simulink library "fmCopterLoiterIndi_lib"  (R2018b)
settings: Solver=VariableStepAuto  StartTime=0.0  StopTime=10.0  RelTol=1e-3
undefined symbols (not defined in the file or in its folder): fm_loiter
libraries: filters_lib x5, indi_lib x3, cntrlAttiRedIndi_lib x1, cntrlPosNdi_lib x1
settings Model: Creator=Ybeyer  LastModifiedBy=yannic
settings SFSimCC: SimUseLocalCustomCode=off
settings RTWCC: RTWUseLocalCustomCode=off
settings CodeAppCC: StateflowObjectComments=on

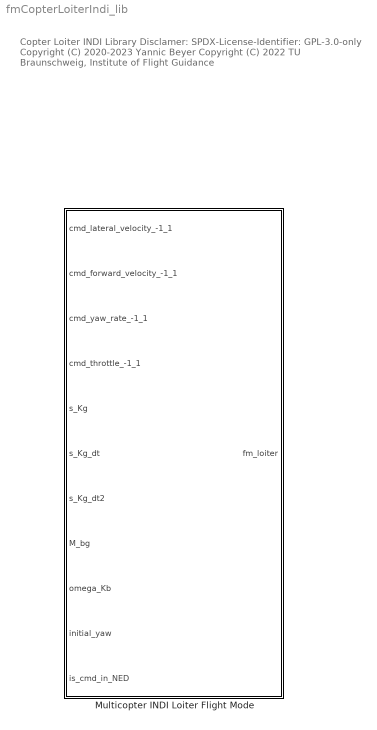
== system fmCopterLoiterIndi_lib ==
  note: Copter Loiter INDI Library
      |
      | Disclamer:
      | SPDX-License-Identifier: GPL-3.0-only
      |
      | Copyright (C) 2020-2023 Yannic Beyer
      | Copyright (C) 2022 TU Braunschweig, Institute of Flight Guidance
  Multicopter INDI Loiter Flight Mode : Subsystem  mask{fm=fm_loiter}
      mask prompts: fm "Copter INDI loiter flight mode parameters struct, see fmCopterLoiterIndi_params_default"
      mask DialogControl DescGroupVar Prompt: Multicopter INDI Loiter Flight Mode
      mask DialogControl DescTextVar Prompt: Loiter flight mode using the reduced attitude controller with INDI.

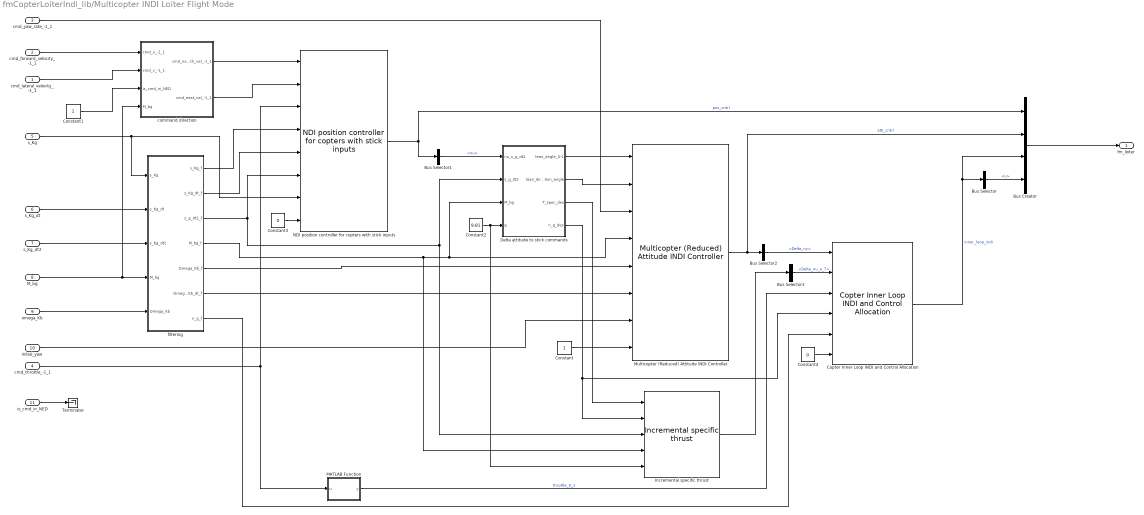
== system fmCopterLoiterIndi_lib/Multicopter INDI Loiter Flight Mode ==
  cmd_lateral_velocity_-1_1 : Inport  SampleTime=fm.ts
  cmd_forward_velocity_-1_1 : Inport  Port=2  SampleTime=fm.ts
  cmd_yaw_rate_-1_1 : Inport  Port=3  SampleTime=fm.ts
  cmd_throttle_-1_1 : Inport  Port=4  SampleTime=fm.ts
  s_Kg : Inport  Port=5  SampleTime=fm.ts
  s_Kg_dt : Inport  Port=6  SampleTime=fm.ts
  s_Kg_dt2 : Inport  Port=7  SampleTime=fm.ts
  M_bg : Inport  Port=8  SampleTime=fm.ts
  omega_Kb : Inport  Port=9  SampleTime=fm.ts
  initial_yaw : Inport  Port=10  SampleTime=fm.ts
  is_cmd_in_NED : Inport  Port=11  SampleTime=fm.ts
  Bus Creator : BusCreator  Inputs=4
  Bus Selector : BusSelector  OutputSignals=u
  Bus Selector1 : BusSelector  OutputSignals=pseudo_control.nu
  Bus Selector2 : BusSelector  OutputSignals=pseudo_control.Delta_ny
  Bus Selector3 : BusSelector  OutputSignals=Delta_nu_a_T
  Constant : Constant
  Constant1 : Constant
  Constant2 : Constant  Value=9.81
  Constant3 : Constant  Value=0
  Constant4 : Constant  Value=0
  Copter Inner Loop INDI and Control Allocation : indi_lib/Copter Inner Loop INDI and Control Allocation  cep=fm.cep  ceb=fm.ceb  ca=fm.ca  mtc=fm.mtc  sflt=fm.sflt  ts=fm.ts
      settings: SourceProductName=LADAC
  Delta attitude to stick commands : Subsystem
  Incremental specific thrust : indi_lib/Incremental specific thrust  leanfreq=fm.atc.rm.leanfreq  leandamp=fm.atc.rm.leandamp  is_enable_checked=off  states_when_enabling=held
      settings: SourceProductName=LADAC
  MATLAB Function : MATLAB Function  TreatAsAtomicUnit=on
  Multicopter (Reduced) Attitude INDI Controller : cntrlAttiRedIndi_lib/Multicopter (Reduced) Attitude INDI Controller  atc=fm.atc  T=fm.mtc + 2./fm.sflt.omega
      settings: SourceProductName=LADAC
  NDI position controller for copters with stick inputs : cntrlPosNdi_lib/NDI position controller for copters with stick inputs  psc=fm.psc  T_inner_loop=2./fm.atc.rm.leanfreq + fm.mtc + 2./fm.sflt.omega  is_enable_checked=off  states_when_enabling=held
      settings: SourceProductName=LADAC
  Terminator : Terminator
  command direction : Subsystem
  filtering : Subsystem
  fm_loiter : Outport  SampleTime=fm.ts
  wires:
  cmd_forward_velocity_-1_1/1 -> command direction/1(cmd_u_-1_1)
  filtering/2(s_Kg_dt_f) -> NDI position controller for copters with stick inputs/5
  filtering/3(s_g_dt2_f) -> NDI position controller for copters with stick inputs/6, Incremental specific thrust/3, Delta attitude to stick commands/2(s_g_dt2)
  cmd_yaw_rate_-1_1/1 -> Multicopter (Reduced) Attitude INDI Controller/3
  Constant/1 -> Multicopter (Reduced) Attitude INDI Controller/8
  filtering/1(s_Kg_f) -> NDI position controller for copters with stick inputs/4
  filtering/5(Omega_Kb_f) -> Multicopter (Reduced) Attitude INDI Controller/5
  NDI position controller for copters with stick inputs/1 -> Bus Creator/1, Bus Selector1/1  "pos_cntrl"
  filtering/4(M_bg_f) -> Incremental specific thrust/4, Multicopter (Reduced) Attitude INDI Controller/4, Delta attitude to stick commands/3(M_bg)
  initial_yaw/1 -> Multicopter (Reduced) Attitude INDI Controller/7
  cmd_lateral_velocity_-1_1/1 -> command direction/2(cmd_v_-1_1)
  Constant1/1 -> command direction/3(is_cmd_in_NED)
  Bus Selector1/1 -> Delta attitude to stick commands/1(nu_s_g_dt2)  "<nu>"
  Bus Creator/1 -> fm_loiter/1
  command direction/1(cmd_north_vel_-1_1) -> NDI position controller for copters with stick inputs/1
  command direction/2(cmd_east_vel_-1_1) -> NDI position controller for copters with stick inputs/2
  is_cmd_in_NED/1 -> Terminator/1
  Multicopter (Reduced) Attitude INDI Controller/1 -> Bus Selector2/1, Bus Creator/2  "atti_cntrl"
  filtering/6(Omega_Kb_dt_f) -> Multicopter (Reduced) Attitude INDI Controller/6
  Delta attitude to stick commands/2(lean_direction_angle) -> Multicopter (Reduced) Attitude INDI Controller/2
  Delta attitude to stick commands/1(lean_angle_0-1) -> Multicopter (Reduced) Attitude INDI Controller/1
  MATLAB Function/1(y) -> Copter Inner Loop INDI and Control Allocation/3  "throttle_0_1"
  Copter Inner Loop INDI and Control Allocation/1 -> Bus Selector/1, Bus Creator/3  "inner_loop_indi"
  cmd_throttle_-1_1/1 -> NDI position controller for copters with stick inputs/3, MATLAB Function/1(u)
  Bus Selector2/1 -> Copter Inner Loop INDI and Control Allocation/1  "<Delta_ny>"
  Constant2/1 -> Incremental specific thrust/5, Delta attitude to stick commands/4(g)
  Bus Selector/1 -> Bus Creator/4  "<u>"
  Incremental specific thrust/1 -> Bus Selector3/1
  Delta attitude to stick commands/3(T_spec_des) -> Incremental specific thrust/1
  Constant3/1 -> NDI position controller for copters with stick inputs/8
  s_Kg/1 -> NDI position controller for copters with stick inputs/7, filtering/1(s_Kg)
  M_bg/1 -> command direction/4(M_bg), filtering/4(M_bg)
  omega_Kb/1 -> filtering/5(Omega_Kb)
  s_Kg_dt2/1 -> filtering/3(s_Kg_dt2)
  s_Kg_dt/1 -> filtering/2(s_Kg_dt)
  filtering/7(n_g_f) -> Copter Inner Loop INDI and Control Allocation/5
  Delta attitude to stick commands/4(n_g_des) -> Copter Inner Loop INDI and Control Allocation/4, Incremental specific thrust/2
  Bus Selector3/1 -> Copter Inner Loop INDI and Control Allocation/2  "<Delta_nu_a_T>"
  Constant4/1 -> Copter Inner Loop INDI and Control Allocation/6

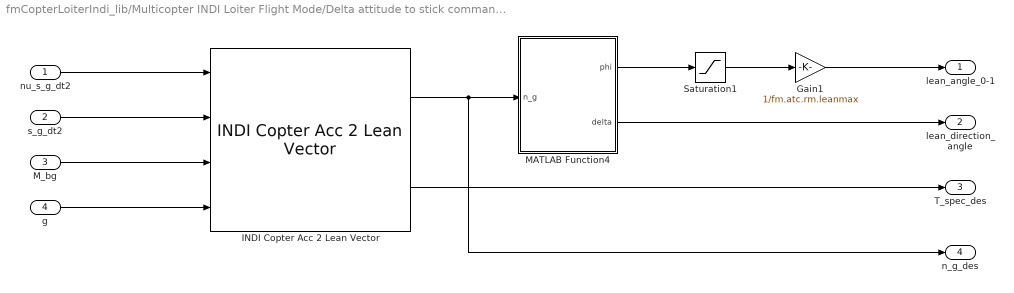
== system fmCopterLoiterIndi_lib/Multicopter INDI Loiter Flight Mode/Delta attitude to stick commands ==
  nu_s_g_dt2 : Inport
  s_g_dt2 : Inport  Port=2
  M_bg : Inport  Port=3
  g : Inport  Port=4
  Gain1 : Gain  Gain=1/fm.atc.rm.leanmax
  INDI Copter Acc 2 Lean Vector : indi_lib/INDI Copter Acc 2 Lean Vector  SystemSampleTime=-1
      settings: SourceProductName=LADAC
  MATLAB Function4 : MATLAB Function  TreatAsAtomicUnit=on
  Saturation1 : Saturate  UpperLimit=fm.atc.rm.leanmax  LowerLimit=0
  lean_angle_0-1 : Outport
  lean_direction_angle : Outport  Port=2
  T_spec_des : Outport  Port=3
  n_g_des : Outport  Port=4
  wires:
  M_bg/1 -> INDI Copter Acc 2 Lean Vector/3
  s_g_dt2/1 -> INDI Copter Acc 2 Lean Vector/2
  g/1 -> INDI Copter Acc 2 Lean Vector/4
  MATLAB Function4/1(phi) -> Saturation1/1
  Saturation1/1 -> Gain1/1
  nu_s_g_dt2/1 -> INDI Copter Acc 2 Lean Vector/1
  Gain1/1 -> lean_angle_0-1/1
  MATLAB Function4/2(delta) -> lean_direction_angle/1
  INDI Copter Acc 2 Lean Vector/1 -> n_g_des/1, MATLAB Function4/1(n_g)
  INDI Copter Acc 2 Lean Vector/2 -> T_spec_des/1

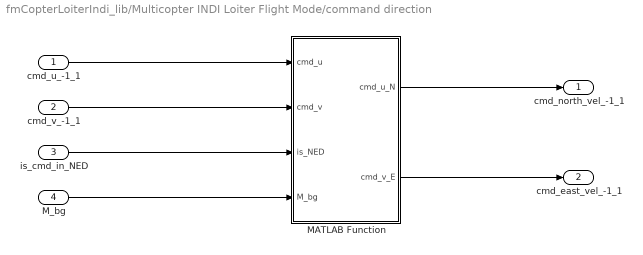
== system fmCopterLoiterIndi_lib/Multicopter INDI Loiter Flight Mode/command direction ==
  cmd_u_-1_1 : Inport
  cmd_v_-1_1 : Inport  Port=2
  is_cmd_in_NED : Inport  Port=3
  M_bg : Inport  Port=4
  MATLAB Function : MATLAB Function  TreatAsAtomicUnit=on
  cmd_north_vel_-1_1 : Outport
  cmd_east_vel_-1_1 : Outport  Port=2
  wires:
  cmd_u_-1_1/1 -> MATLAB Function/1(cmd_u)
  cmd_v_-1_1/1 -> MATLAB Function/2(cmd_v)
  is_cmd_in_NED/1 -> MATLAB Function/3(is_NED)
  MATLAB Function/1(cmd_u_N) -> cmd_north_vel_-1_1/1
  MATLAB Function/2(cmd_v_E) -> cmd_east_vel_-1_1/1
  M_bg/1 -> MATLAB Function/4(M_bg)

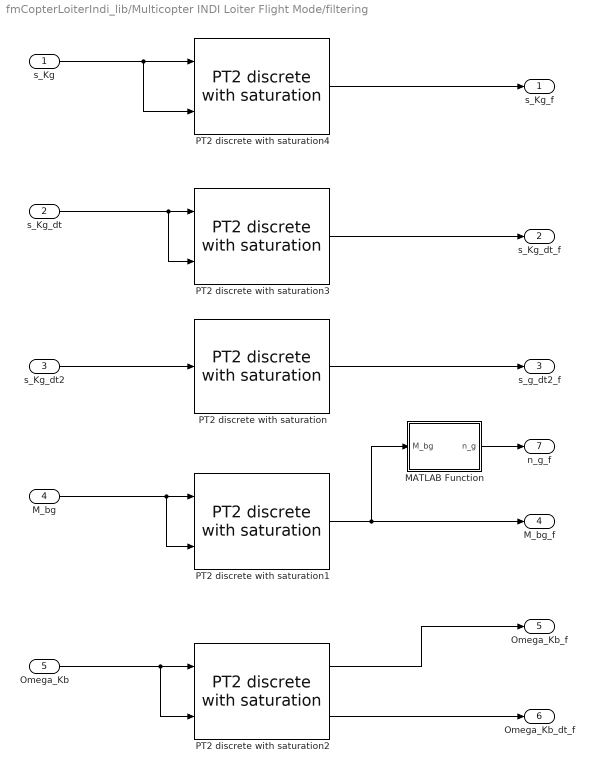
== system fmCopterLoiterIndi_lib/Multicopter INDI Loiter Flight Mode/filtering ==
  s_Kg : Inport
  s_Kg_dt : Inport  Port=2
  s_Kg_dt2 : Inport  Port=3
  M_bg : Inport  Port=4
  Omega_Kb : Inport  Port=5
  MATLAB Function : MATLAB Function  TreatAsAtomicUnit=on
  PT2 discrete with saturation : filters_lib/PT2 discrete with saturation  param_src=internal  omega=fm.sflt.omega  d=fm.sflt.D  x_dt2_max=inf  x_dt2_min=-inf  x_dt_max=inf  x_dt_min=-inf  x_max=inf  x_min=-inf  y_0_src=internal  x_init=0  y_dt_0_src=internal  x_dt_init=0  is_y_dt_checked=off  is_y_dt2_checked=off
      settings: SourceProductName=LADAC
  PT2 discrete with saturation1 : filters_lib/PT2 discrete with saturation  param_src=internal  omega=fm.sflt.omega  d=fm.sflt.D  x_dt2_max=inf  x_dt2_min=-inf  x_dt_max=inf  x_dt_min=-inf  x_max=inf  x_min=-inf  y_0_src=external  x_init=0  y_dt_0_src=internal  x_dt_init=0  is_y_dt_checked=off  is_y_dt2_checked=off
      settings: SourceProductName=LADAC
  PT2 discrete with saturation2 : filters_lib/PT2 discrete with saturation  param_src=internal  omega=fm.sflt.omega  d=fm.sflt.D  x_dt2_max=inf  x_dt2_min=-inf  x_dt_max=inf  x_dt_min=-inf  x_max=inf  x_min=-inf  y_0_src=external  x_init=0  y_dt_0_src=internal  x_dt_init=0  is_y_dt_checked=on  is_y_dt2_checked=off
      settings: SourceProductName=LADAC
  PT2 discrete with saturation3 : filters_lib/PT2 discrete with saturation  param_src=internal  omega=fm.sflt.omega  d=fm.sflt.D  x_dt2_max=inf  x_dt2_min=-inf  x_dt_max=inf  x_dt_min=-inf  x_max=inf  x_min=-inf  y_0_src=external  x_init=0  y_dt_0_src=internal  x_dt_init=0  is_y_dt_checked=off  is_y_dt2_checked=off
      settings: SourceProductName=LADAC
  PT2 discrete with saturation4 : filters_lib/PT2 discrete with saturation  param_src=internal  omega=fm.sflt.omega  d=fm.sflt.D  x_dt2_max=inf  x_dt2_min=-inf  x_dt_max=inf  x_dt_min=-inf  x_max=inf  x_min=-inf  y_0_src=external  x_init=0  y_dt_0_src=internal  x_dt_init=0  is_y_dt_checked=off  is_y_dt2_checked=off
      settings: SourceProductName=LADAC
  s_Kg_f : Outport
  s_Kg_dt_f : Outport  Port=2
  s_g_dt2_f : Outport  Port=3
  M_bg_f : Outport  Port=4
  Omega_Kb_f : Outport  Port=5
  Omega_Kb_dt_f : Outport  Port=6
  n_g_f : Outport  Port=7
  wires:
  PT2 discrete with saturation2/2 -> Omega_Kb_dt_f/1
  Omega_Kb/1 -> PT2 discrete with saturation2/2, PT2 discrete with saturation2/1
  PT2 discrete with saturation2/1 -> Omega_Kb_f/1
  M_bg/1 -> PT2 discrete with saturation1/2, PT2 discrete with saturation1/1
  PT2 discrete with saturation/1 -> s_g_dt2_f/1
  s_Kg_dt2/1 -> PT2 discrete with saturation/1
  PT2 discrete with saturation3/1 -> s_Kg_dt_f/1
  s_Kg_dt/1 -> PT2 discrete with saturation3/2, PT2 discrete with saturation3/1
  PT2 discrete with saturation4/1 -> s_Kg_f/1
  s_Kg/1 -> PT2 discrete with saturation4/1, PT2 discrete with saturation4/2
  PT2 discrete with saturation1/1 -> MATLAB Function/1(M_bg), M_bg_f/1
  MATLAB Function/1(n_g) -> n_g_f/1

== matlab function fmCopterLoiterIndi_lib/Multicopter INDI Loiter Flight Mode/command direction/MATLAB Function ==
  data: cmd_u input; cmd_u_N output; cmd_v input; is_NED input; cmd_v_E output; M_bg input
function [cmd_u_N,cmd_v_E] = fcn( cmd_u, cmd_v, is_NED, M_bg )

if is_NED
    cmd_u_N = cmd_u;
    cmd_v_E = cmd_v;
else
    EulerAngle = dcm2Euler(M_bg);
    yaw = EulerAngle(3);
    M_NED_FRD = euler2Dcm([0;0;yaw])';
    cmd_V_NED = M_NED_FRD * [ cmd_u; cmd_v; 0 ];
    cmd_u_N = cmd_V_NED(1);
    cmd_v_E = cmd_V_NED(2);
end

end

== matlab function fmCopterLoiterIndi_lib/Multicopter INDI Loiter Flight Mode/filtering/MATLAB Function ==
  data: M_bg input; n_g output
function n_g = dcm2LeanVector( M_bg )
n_g = dcm2LeanVector( M_bg );
end

== matlab function fmCopterLoiterIndi_lib/Multicopter INDI Loiter Flight Mode/Delta attitude to stick commands/MATLAB Function4 ==
  data: n_g input; phi output; delta output
function [phi,delta] = leanVector2LeanAngles(n_g)
[phi,delta] = leanVector2LeanAngles(n_g);
end

== matlab function fmCopterLoiterIndi_lib/Multicopter INDI Loiter Flight Mode/MATLAB Function ==
  data: u input; y output
function y = fcn(u)
y = 0.5*u+0.5;
